simulink model "Complete_SAD_model"  (R2025b)
settings: Solver=ode4  StartTime=0.0  StopTime=10  FixedStep=0.01  RelTol=1e-3
values from neighbouring files (symbols this model uses):
  A = eye(3)    [Initial_condition.m]
  a_pink = exp(-2*pi*fc_pink*Ts_m*k_pink)    [Initial_condition.m]
  acc = deg2rad(0.5*randn)    [Initial_condition.m]
  Ap = eye(3)    [Initial_condition.m]
  D = 500*10^-12    (= 5e-10)    [Initial_condition.m]
  delay = 1    [Initial_condition.m]
  inv_Ir = inv(Ir)    [Initial_condition.m]
  Ir = diag([Irx,Iry,Irz])    [Initial_condition.m]
  J_B = diag([Ix,Iy,Iz])    [Initial_condition.m]
  m = [0.01; 0.01; 0.01]    [Initial_condition.m]
  m_max = [0.65; 0.65; 0.5]    [Initial_condition.m]
  Mr_max = [0.01; 0.01; 0.01]    [Initial_condition.m]
  mu_earth = 398600.433    [Initial_condition.m]
  mu_sun = 132712440017.987    (= 132712440018)    [Initial_condition.m]
  non_ort = deg2rad(-1+2*rand)    [Initial_condition.m]
  omega0 = [wx;wy;wz]    [Initial_condition.m]
  rES0_ECI = [0 AU 0]    [Initial_condition.m]
  seed = 0    [Initial_condition.m]
  sigma = (2*pi/60)/3    (= 0.0349065850399)    [Initial_condition.m]
  Ts_m = 1/f_m    (= 0.1)    [Initial_condition.m]
  Ts_ss = 1/f_ss    (= 0.1)    [Initial_condition.m]
  vES0_ECI = [(-sqrt(mu_sun/norm(rES0_ECI))) 0 0 ]    [Initial_condition.m]
  w_max = [250; 250; 250]    [Initial_condition.m]
undefined symbols (not defined in the file or in its folder): dspblkCoreblockFVToolHelper, gcbh, K, r0_ECI, v0_ECI
libraries: matrix_library x15, dspmathops x3, dspfdesign x3, vrlib x2
(part 1 of 3)
settings Model: Creator=Utente  LastModifiedBy=loren

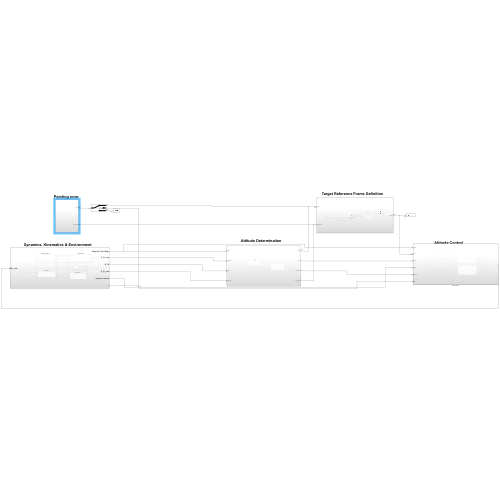
[thumbnail: Simulink's stored preview of the top-level diagram]
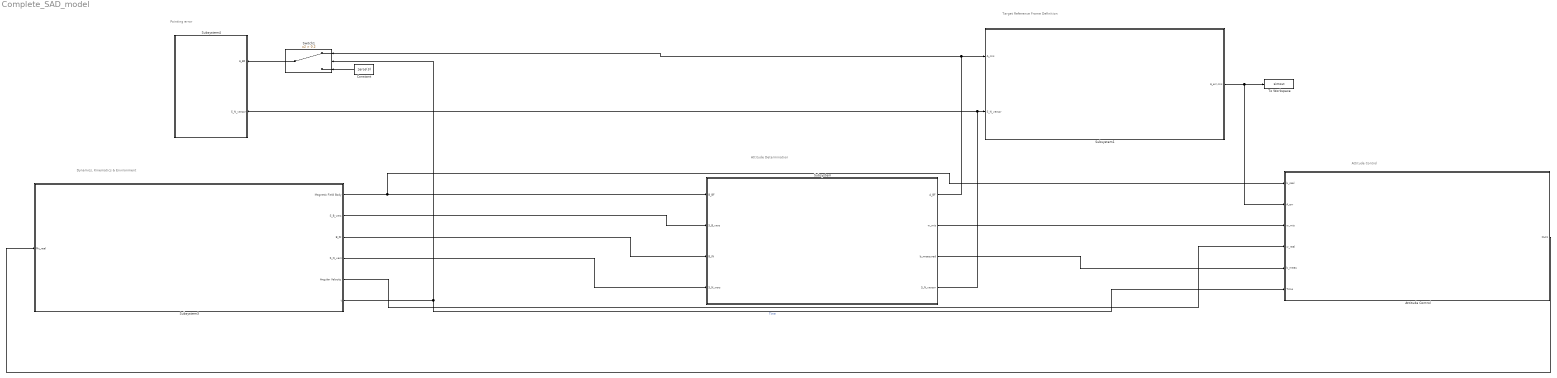
== system Complete_SAD_model ==
  note: Dynamics, Kinematics & Environment
  note: Attitude Determination
  note: Attitude Control
  note: Target Reference Frame Definition
  note: Pointing error
  Attitude Control : Subsystem
  Constant : Constant  Value=zeros(3)
  Subsystem : Subsystem
  Subsystem1 : Subsystem
  Subsystem3 : Subsystem
  Subsystem4 : Subsystem
  Switch1 : Switch  Criteria=u2 > Threshold  Threshold=0.2  SaturateOnIntegerOverflow=off  InputSameDT=off
  To Workspace : ToWorkspace  VariableName=simout  SaveFormat=Timeseries  SampleTime=-1
  wires:
  Subsystem3/1(Magnetic Field Body) -> Attitude Control/1(b_real), Subsystem/1(B_BF)
  Subsystem3/2(S_B_vers) -> Subsystem/2(S_B_vers)
  Subsystem3/3(B_IN) -> Subsystem/3(B_IN)
  Subsystem3/4(S_N_vers) -> Subsystem/4(S_N_vers)
  Subsystem/1(A_BF) -> Switch1/1, Subsystem1/1(A_mis)
  Subsystem/2(w_mis) -> Attitude Control/3(w_mis)
  Subsystem3/5(Angular Velocity) -> Attitude Control/4(w_real)
  Subsystem/3(b_measured) -> Attitude Control/5(b_meas)
  Subsystem3/6(t) -> Switch1/2, Attitude Control/6(Time)  "Time"
  Attitude Control/1(Out1) -> Subsystem3/1(Mc_real)
  Subsystem/4(S_N_versor) -> Subsystem4/2(S_N_versor), Subsystem1/2(S_N_versor)
  Subsystem1/1(A_err,mis) -> To Workspace/1, Attitude Control/2(A_err)
  Switch1/1 -> Subsystem4/1(A_BF)
  Constant/1 -> Switch1/3

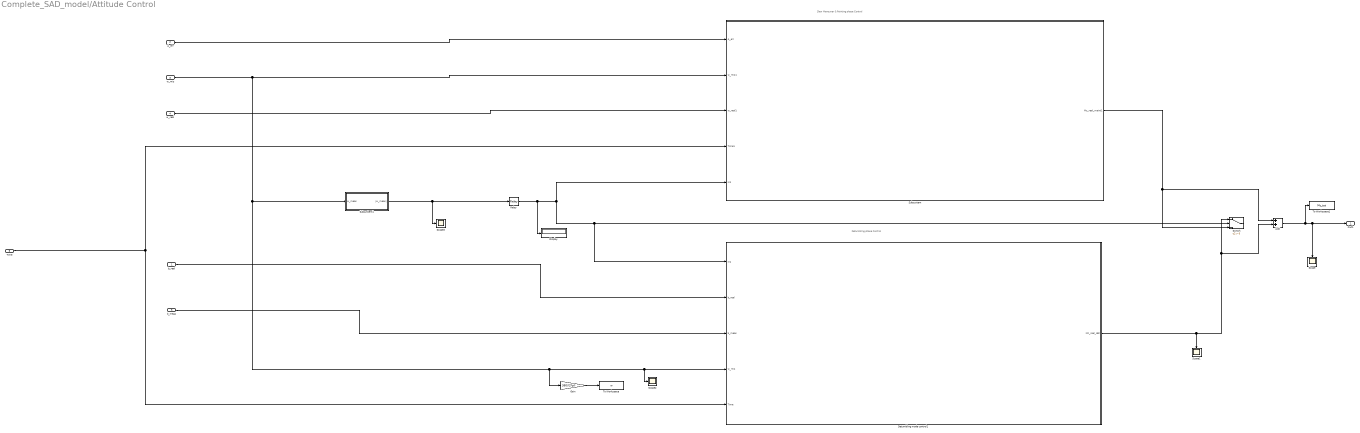
== system Complete_SAD_model/Attitude Control ==
  note: Detumbling phase Control
  note: Slew Manouver & Pointing phase Control
  b_real : Inport
  A_err : Inport  Port=2
  w_mis : Inport  Port=3
  w_real : Inport  Port=4
  b_meas : Inport  Port=5
  Time : Inport  Port=6
  Add : Sum
  Detumbling mode control1 : Subsystem
  Display : Display
  Gain : Gain  Gain=360/(2*pi)
  Relay : Relay  OnSwitchValue=0.15  OffSwitchValue=deg2rad(5)
  Scope{,1..3} (4 alike) : Scope
      Scope settings: ActiveDisplayYMinimum=-0.00066406553970955529  ActiveDisplayYMaximum=0.000676333066590346  DataLoggingVariableName=ScopeData20
      Scope1 settings: ActiveDisplayYMinimum=-0.000218043993955084  ActiveDisplayYMaximum=0.00024658945561407578  DataLoggingVariableName=ScopeData24
      Scope2 settings: ActiveDisplayYMinimum=-0.80919246331980188  ActiveDisplayYMaximum=0.81042984032750753  DataLoggingVariableName=ScopeData32
      Scope3 settings: ActiveDisplayYMinimum=0.021025794822100707  ActiveDisplayYMaximum=0.38469575455597654  DataLoggingVariableName=ScopeData37
  Subsystem : Subsystem
  Subsystem1 : Subsystem
  Switch : Switch  Criteria=u2 > Threshold  SaturateOnIntegerOverflow=off  InputSameDT=off
  To Workspace : ToWorkspace  VariableName=w  SaveFormat=Timeseries  SampleTime=-1
  To Workspace1 : ToWorkspace  VariableName=Mc_tot  SampleTime=-1
  Out1 : Outport
  wires:
  b_real/1 -> Detumbling mode control1/2(b_real)
  Detumbling mode control1/1(Mc_real_det) -> Scope1/1, Add/2, Switch/1
  Time/1 -> Subsystem/4(Time1), Detumbling mode control1/5(Time)
  b_meas/1 -> Detumbling mode control1/3(b_meas)
  w_mis/1 -> Subsystem1/1(w_meas), Gain/1, Scope2/1, Detumbling mode control1/4(w_mis), Subsystem/2(w_mis1)
  A_err/1 -> Subsystem/1(A_err)
  w_real/1 -> Subsystem/3(w_real1)
  Subsystem1/1(|w_meas|) -> Scope3/1, Relay/1
  Relay/1 -> Display/1, Subsystem/5(In1), Detumbling mode control1/1(In1), Switch/2
  Subsystem/1(Mc_real_maint1) -> Add/1, Switch/3
  Add/1 -> To Workspace1/1, Scope/1, Out1/1
  Gain/1 -> To Workspace/1

== system Complete_SAD_model/Subsystem ==
  note: Determination Algorithm
  note: Sensors
  B_BF : Inport
  S_B_vers : Inport  Port=2
  B_IN : Inport  Port=3
  S_N_vers : Inport  Port=4
  Determination Algorithm : Subsystem
  Scope : Scope
      settings: ActiveDisplayYMinimum=-1.125  ActiveDisplayYMaximum=0.12499999999999997  DataLoggingVariableName=ScopeData39
  Scope1 : Scope
      settings: ActiveDisplayYMinimum=-7.094188804581898E-5  ActiveDisplayYMaximum=5.8924288015728448E-5  DataLoggingVariableName=ScopeData40
  Subsystem2 : Subsystem
  A_BF : Outport
  w_mis : Outport  Port=2
  b_measured : Outport  Port=3
  S_N_versor : Outport  Port=4
  wires:
  S_B_vers/1 -> Subsystem2/2(S_B_vers)
  S_N_vers/1 -> Scope/1, S_N_versor/1, Determination Algorithm/4(S_N_vers)
  Subsystem2/1(b_measured) -> Determination Algorithm/2(b_measured), b_measured/1
  Determination Algorithm/1(A_BF) -> A_BF/1
  Subsystem2/2(S_B_measured) -> Determination Algorithm/1(S_B_measured)
  Determination Algorithm/2(w_mis) -> w_mis/1
  B_BF/1 -> Subsystem2/1(B_BF)
  B_IN/1 -> Scope1/1, Determination Algorithm/3(B_IN)

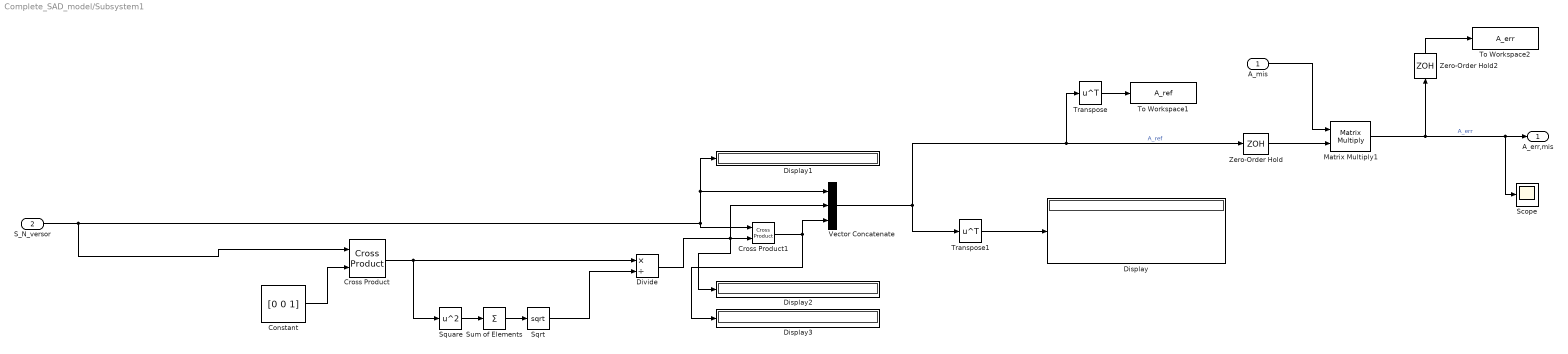
== system Complete_SAD_model/Subsystem1 ==
  A_mis : Inport
  S_N_versor : Inport  Port=2
  Constant : Constant  Value=[0 0 1]
  Cross Product : matrix_library/Cross Product
  Cross Product1 : matrix_library/Cross Product
  Display{,1..3} (4 alike) : Display
  Divide : Product  Inputs=*/
  Matrix Multiply1 : Product  Multiplication=Matrix(*)
  Scope : Scope
      settings: ActiveDisplayYMinimum=-1.0313451799509168  ActiveDisplayYMaximum=2.1593552960699949  DataLoggingVariableName=ScopeData36
  Sqrt : Sqrt
  Square : Math  Operator=square
  Sum of Elements : Sum  Inputs=+
  To Workspace1 : ToWorkspace  VariableName=A_ref  SampleTime=-1
  To Workspace2 : ToWorkspace  VariableName=A_err  SampleTime=-1
  Transpose : Math  Operator=transpose
  Transpose1 : Math  Operator=transpose
  Vector Concatenate : Concatenate  NumInputs=3  Mode=Multidimensional array  ConcatenateDimension=2
  Zero-Order Hold : ZeroOrderHold  SampleTime=0.1
  Zero-Order Hold2 : ZeroOrderHold  SampleTime=0.01
  A_err,mis : Outport
  wires:
  Square/1 -> Sum of Elements/1
  Zero-Order Hold/1 -> Matrix Multiply1/2
  Cross Product1/1 -> Vector Concatenate/3, Display3/1
  Sqrt/1 -> Divide/2
  Transpose/1 -> To Workspace1/1
  Matrix Multiply1/1 -> Zero-Order Hold2/1, Scope/1, A_err,mis/1  "A_err"
  Sum of Elements/1 -> Sqrt/1
  Vector Concatenate/1 -> Transpose1/1, Transpose/1, Zero-Order Hold/1  "A_ref"
  A_mis/1 -> Matrix Multiply1/1
  Zero-Order Hold2/1 -> To Workspace2/1
  Divide/1 -> Vector Concatenate/2, Display2/1, Cross Product1/2
  Cross Product/1 -> Divide/1, Square/1
  Constant/1 -> Cross Product/2
  S_N_versor/1 -> Cross Product/1, Vector Concatenate/1, Display1/1, Cross Product1/1
  Transpose1/1 -> Display/1

== system Complete_SAD_model/Subsystem3 ==
  note: Perturbations
  note: Dynamics
  note: Kinematics
  note: Orbit Propagation
  Mc_real : Inport
  " Attitude Dynamics" : Subsystem
  Attitude Kinematics  with orthonormalization : Subsystem
  Constant : Constant  Value=J_B
  Disturbance Torques : Subsystem
  Divide : Product  Inputs=*/
  MatrixMultiply : Product  Multiplication=Matrix(*)
  Orbita Propagation1 : Subsystem
  Scope : Scope
      settings: ActiveDisplayYMinimum=-0.0048523047678160009  ActiveDisplayYMaximum=0.00453129877837137  DataLoggingVariableName=ScopeData51
  Vector_Norm : Subsystem
  Magnetic Field Body : Outport
  S_B_vers : Outport  Port=2
  B_IN : Outport  Port=3
  S_N_vers : Outport  Port=4
  Angular Velocity : Outport  Port=5
  t : Outport  Port=6
  wires:
  Mc_real/1 -> " Attitude Dynamics"/3(Mc_real), Scope/1
  Disturbance Torques/4(t) -> t/1
  MatrixMultiply/1 -> S_B_vers/1
  Divide/1 -> MatrixMultiply/2, S_N_vers/1
  Vector_Norm/1(norm) -> Divide/2  "Position_Norm"
  Orbita Propagation1/4(r_SC/S) -> Vector_Norm/1(vector), Divide/1
  Disturbance Torques/3(B_IN) -> B_IN/1
  Disturbance Torques/2(Magnetic Field Body) -> Magnetic Field Body/1
  Attitude Kinematics  with orthonormalization/2(A_B | L) -> Disturbance Torques/5(A_B | L)
  Orbita Propagation1/2(h vector) -> Attitude Kinematics  with orthonormalization/3(h vector)
  Constant/1 -> Disturbance Torques/4("Matrix of Inertia "), " Attitude Dynamics"/1(Inertia Matrix)
  Orbita Propagation1/1("Norm of Position Spacecraft - Earth ") -> Disturbance Torques/1(Norm Position)
  Orbita Propagation1/3(Versore Posizione) -> Disturbance Torques/2(versore_Posizione), Attitude Kinematics  with orthonormalization/2(Versore Posizione)
  Disturbance Torques/1(Disturbance) -> " Attitude Dynamics"/2(Disturbo)
  " Attitude Dynamics"/1(Angular Velocity) -> Angular Velocity/1, Attitude Kinematics  with orthonormalization/1(Angular Velocity)
  Attitude Kinematics  with orthonormalization/1(Direction Cosine Matrix) -> MatrixMultiply/1, Disturbance Torques/3(DCM)

== system Complete_SAD_model/Subsystem4 ==
  A_BF : Inport
  S_N_versor : Inport  Port=2
  Acos : Trigonometry  Operator=acos
  Dot Product : DotProduct  OutDataTypeStr=Inherit: Inherit via internal rule
  Gain : Gain  Gain=360/(2*pi)
  Normalization : dspmathops/Normalization  NormType=2-norm  Bias=1e-10  NormOver=Each column  Dimension=1  roundingMode=Floor  overflowMode=off  accumDataTypeStr=Inherit: Same as product output  accumLastDataTypeStr=Inherit: Same as product output  outputDataTypeStr=Inherit: Same as product output  outputMin=[]  outputMax=[]  outputLastDataTypeStr=Inherit: Same as product output
  Normalization1 : dspmathops/Normalization  NormType=2-norm  Bias=1e-10  NormOver=Each column  Dimension=1  roundingMode=Floor  overflowMode=off  accumDataTypeStr=Inherit: Same as product output  accumLastDataTypeStr=Inherit: Same as product output  outputDataTypeStr=Inherit: Same as product output  outputMin=[]  outputMax=[]  outputLastDataTypeStr=Inherit: Same as product output
  Scope : Scope
      settings: ActiveDisplayYMinimum=-22.453635883732677  ActiveDisplayYMaximum=202.09419906568513  DataLoggingVariableName=ScopeData71
  Selector : Selector  NumberOfDimensions=2  InputPortWidth=3  IndexOptions=Index vector (dialog),Index vector (dialog)  Indices=1,1  OutputSizes=1,1
  Selector2 : Selector  NumberOfDimensions=2  InputPortWidth=3  IndexOptions=Index vector (dialog),Index vector (dialog)  Indices=1,2  OutputSizes=1,1
  Selector4 : Selector  NumberOfDimensions=2  InputPortWidth=3  IndexOptions=Index vector (dialog),Index vector (dialog)  Indices=1,3  OutputSizes=1,1
  To Workspace : ToWorkspace  VariableName=pointing_error  SampleTime=-1
  Vector Concatenate : Concatenate  NumInputs=3
  wires:
  Selector2/1 -> Vector Concatenate/2  "a12"
  Selector/1 -> Vector Concatenate/1  "a11"
  Selector4/1 -> Vector Concatenate/3  "a13"
  A_BF/1 -> Selector/1, Selector4/1, Selector2/1
  Vector Concatenate/1 -> Normalization1/1  "x_BF"
  S_N_versor/1 -> Normalization/1
  Normalization/1 -> Dot Product/1
  Normalization1/1 -> Dot Product/2
  Dot Product/1 -> Acos/1
  Acos/1 -> Gain/1
  Gain/1 -> Scope/1, To Workspace/1

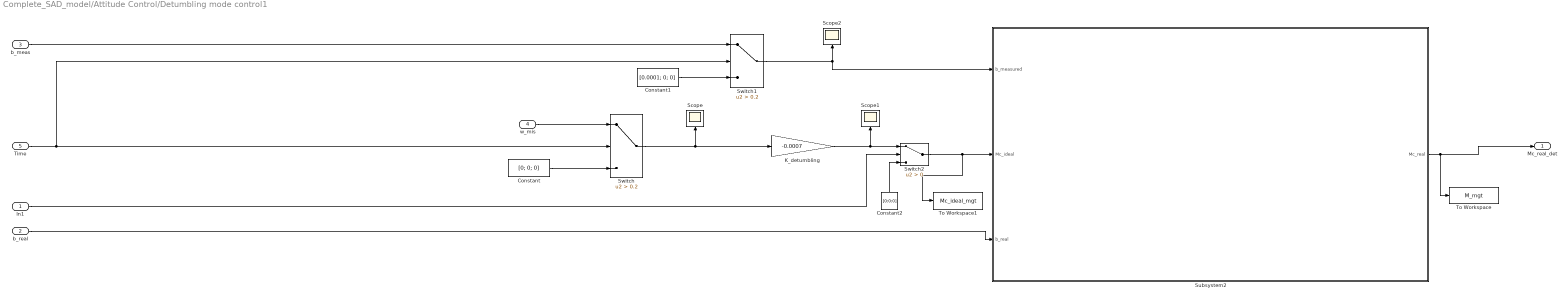
== system Complete_SAD_model/Attitude Control/Detumbling mode control1 ==
  In1 : Inport
  b_real : Inport  Port=2
  b_meas : Inport  Port=3
  w_mis : Inport  Port=4
  Time : Inport  Port=5
  Constant : Constant  Value=[0; 0; 0]
  Constant1 : Constant  Value=[0.0001; 0; 0]
  Constant2 : Constant  Value=[0;0;0]
  K_detumbling : Gain  Gain=-0.0007
  Scope : Scope
      settings: ActiveDisplayYMinimum=-0.83224888402197306  ActiveDisplayYMaximum=0.87185250448284746  DataLoggingVariableName=ScopeData3
  Scope1 : Scope
      settings: ActiveDisplayYMinimum=-0.001056362749452055  ActiveDisplayYMaximum=0.0010198107488302737  DataLoggingVariableName=ScopeData17
  Scope2 : Scope
      settings: ActiveDisplayYMinimum=-0.00021732143270324306  ActiveDisplayYMaximum=0.00011510450718215886  DataLoggingVariableName=ScopeData5
  Subsystem2 : Subsystem
  Switch : Switch  Criteria=u2 > Threshold  Threshold=0.2  SaturateOnIntegerOverflow=off  InputSameDT=off
  Switch1 : Switch  Criteria=u2 > Threshold  Threshold=0.2  SaturateOnIntegerOverflow=off  InputSameDT=off
  Switch2 : Switch  Criteria=u2 > Threshold  SaturateOnIntegerOverflow=off  InputSameDT=off
  To Workspace : ToWorkspace  VariableName=M_mgt  SampleTime=-1
  To Workspace1 : ToWorkspace  VariableName=Mc_ideal_mgt  SampleTime=-1
  Mc_real_det : Outport
  wires:
  b_meas/1 -> Switch1/1
  Constant/1 -> Switch/3
  Constant1/1 -> Switch1/3
  w_mis/1 -> Switch/1
  K_detumbling/1 -> Switch2/1, Scope1/1
  Switch1/1 -> Scope2/1, Subsystem2/1(b_measured)
  Switch/1 -> K_detumbling/1, Scope/1
  Time/1 -> Switch1/2, Switch/2
  b_real/1 -> Subsystem2/3(b_real)
  In1/1 -> Switch2/2
  Constant2/1 -> Switch2/3
  Switch2/1 -> To Workspace1/1, Subsystem2/2(Mc_ideal)
  Subsystem2/1(Mc_real) -> To Workspace/1, Mc_real_det/1

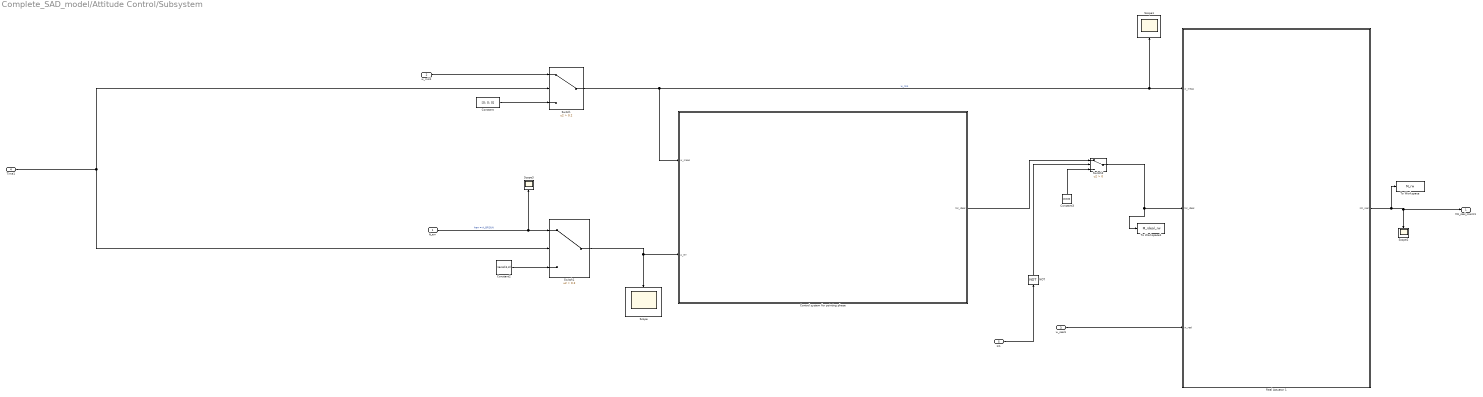
== system Complete_SAD_model/Attitude Control/Subsystem ==
  A_err : Inport
  w_mis1 : Inport  Port=2
  w_real1 : Inport  Port=3
  Time1 : Inport  Port=4
  In1 : Inport  Port=5
  Constant : Constant  Value=[0; 0; 0]
  Constant2 : Constant  Value=zeros(3,3)
  Constant3 : Constant  Value=[0;0;0]
  Control system for pointing phase : Subsystem
  NOT : Logic  Operator=NOT  IconShape=distinctive  AllPortsSameDT=off  OutDataTypeStr=boolean
  Real Actuator 1 : Subsystem
  Scope{,1..3} (4 alike) : Scope
      Scope settings: ActiveDisplayYMinimum=0.51490356419952588  ActiveDisplayYMaximum=1.1113602060789165  DataLoggingVariableName=ScopeData21
      Scope1 settings: ActiveDisplayYMinimum=-0.040624605457754565  ActiveDisplayYMaximum=0.040024288147769135  DataLoggingVariableName=ScopeData22
      Scope2 settings: ActiveDisplayYMinimum=-0.0019839698452016928  ActiveDisplayYMaximum=0.0020094703349881932  DataLoggingVariableName=ScopeData23
      Scope3 settings: DataLoggingVariableName=ScopeData28
  Switch : Switch  Criteria=u2 > Threshold  Threshold=0.2  SaturateOnIntegerOverflow=off  InputSameDT=off
  Switch1 : Switch  Criteria=u2 > Threshold  Threshold=0.2  SaturateOnIntegerOverflow=off  InputSameDT=off
  Switch2 : Switch  Criteria=u2 > Threshold  SaturateOnIntegerOverflow=off  InputSameDT=off
  To Workspace : ToWorkspace  VariableName=M_rw  SampleTime=-1
  To Workspace1 : ToWorkspace  VariableName=M_ideal_rw  SampleTime=-1
  Mc_real_maint1 : Outport
  wires:
  In1/1 -> NOT/1
  Time1/1 -> Switch1/2, Switch/2
  A_err/1 -> Switch1/1, Scope3/1  "Aerr = A_BF/SUN"
  Constant/1 -> Switch/3
  w_real1/1 -> Real Actuator 1/3(w_real)
  Switch1/1 -> Scope/1, Control system for pointing phase/2(A_err)
  w_mis1/1 -> Switch/1
  Switch/1 -> Real Actuator 1/1(w_meas), Scope1/1, Control system for pointing phase/1(w_meas)  "w_mis"
  Constant2/1 -> Switch1/3
  Control system for pointing phase/1(Mc_ideal) -> Switch2/1
  NOT/1 -> Switch2/2
  Constant3/1 -> Switch2/3
  Switch2/1 -> To Workspace1/1, Real Actuator 1/2(Mc_ideal)
  Real Actuator 1/1(Mc_real) -> To Workspace/1, Mc_real_maint1/1, Scope2/1

== system Complete_SAD_model/Attitude Control/Subsystem1 ==
  w_meas : Inport
  Sqrt : Sqrt
  Square : Math  Operator=square
  Sum of Elements : Sum  Inputs=+
  |w_meas| : Outport
  wires:
  w_meas/1 -> Square/1
  Sqrt/1 -> |w_meas|/1
  Square/1 -> Sum of Elements/1
  Sum of Elements/1 -> Sqrt/1

== system Complete_SAD_model/Subsystem/Determination Algorithm ==
  S_B_measured : Inport
  b_measured : Inport  Port=2
  B_IN : Inport  Port=3
  S_N_vers : Inport  Port=4
  ALGEBRAIC METHOD for ATTITUDE DETERMINATION 1 : Subsystem
  Angular velocity determination1 : Subsystem
  Scope{,1..5} (6 alike) : Scope
      Scope settings: ActiveDisplayYMinimum=-1  ActiveDisplayYMaximum=1  DataLoggingVariableName=ScopeData53
      Scope1 settings: ActiveDisplayYMinimum=-2.7577259976289361  ActiveDisplayYMaximum=2.8520572470875512  DataLoggingVariableName=ScopeData57
      Scope2 settings: DataLoggingVariableName=ScopeData58
      Scope3 settings: DataLoggingVariableName=ScopeData59
      Scope4 settings: DataLoggingVariableName=ScopeData60
      Scope5 settings: DataLoggingVariableName=ScopeData61
  A_BF : Outport
  w_mis : Outport  Port=2
  wires:
  ALGEBRAIC METHOD for ATTITUDE DETERMINATION 1/1(A_mis) -> A_BF/1, Scope/1, Angular velocity determination1/1(A_mis)  "A_BF"
  S_B_measured/1 -> Scope4/1, ALGEBRAIC METHOD for ATTITUDE DETERMINATION 1/2(S_B_measured)
  S_N_vers/1 -> Scope2/1, ALGEBRAIC METHOD for ATTITUDE DETERMINATION 1/4(S_N_vers)
  B_IN/1 -> Scope3/1, ALGEBRAIC METHOD for ATTITUDE DETERMINATION 1/3(B_IN)
  Angular velocity determination1/1(w_mis) -> Scope1/1, w_mis/1  "w_mis"
  b_measured/1 -> Scope5/1, ALGEBRAIC METHOD for ATTITUDE DETERMINATION 1/1(b_measured)

== system Complete_SAD_model/Subsystem/Subsystem2 ==
  note: Magnetometer
  note: Sun Sensor
  B_BF : Inport
  S_B_vers : Inport  Port=2
  MAGNETOMETER : Subsystem
  SUN SENSOR : Subsystem
      settings: PortSchema="{\"entries\":[{\"content\":{\"sides\":[{\"content\":{\"connectorIds\":[\"In1\"]},\"type\":\"ConnectorPlacement.EquallySpacedRectSide\",\"uuid\":\"3307fc53-f976-44c0-b732-30d51e7de2d2\"},{\"content\":{\"connectorIds\":[\"Out1\"],\"side\":\"RIGHT\"},\"type\":\"ConnectorPlacement.EquallySpacedRectSide\",\"uuid\":\"dd005eaf-9f48-4a06-9a65-62dab91bec2a\"},{\"content\":{\"side\":\"TOP\"},\"type\":\"ConnectorPlacement.EquallySpacedRectSide\",\"uuid\":\"b87f2816-b76f-4367-9475-2b3209047cf2\"},{\"content\":{\"connectorIds\":[\"Out2\"],\"side\":\"BOTTOM\"},\"type\":\"ConnectorPlacement.EquallySpacedRectSide\",\"uuid\":\"f1acf421-c567-4b56-8ca9-be9bc34615ea\"}]},\"type\":\"ConnectorPlacement.EquallySpacedConnector\",\"uuid\":\"0af9b085-f877-4503-8798-90c3da9edf65\"}],\"packageUris\":[\"http://schema.mathworks.com/mf0/Connector/R2020b\"],\"version\":\"1.0\"}"
  b_measured : Outport
  S_B_measured : Outport  Port=2
  wires:
  S_B_vers/1 -> SUN SENSOR/1(S_B_vers)
  B_BF/1 -> MAGNETOMETER/1(B_BF)
  SUN SENSOR/1(S_B_measured) -> S_B_measured/1
  MAGNETOMETER/1(b_measured) -> b_measured/1

== system Complete_SAD_model/Subsystem3/ Attitude Dynamics ==
  Inertia Matrix : Inport
  Disturbo : Inport  Port=2
  Mc_real : Inport  Port=3
  Add : Sum  Inputs=+++
  Cross Product : matrix_library/Cross Product
  Gain : Gain  Gain=inv(J_B)  Multiplication=Matrix(K*u)
  Integrator : Integrator  InitialCondition=omega0
  Product : Product  Multiplication=Matrix(*)
  Scope : Scope
      settings: ActiveDisplayYMinimum=-1  ActiveDisplayYMaximum=1  DataLoggingVariableName=ScopeData25
  Scope1 : Scope
      settings: ActiveDisplayYMinimum=-1  ActiveDisplayYMaximum=1  DataLoggingVariableName=ScopeData26
  Scope2 : Scope
      settings: ActiveDisplayYMinimum=-1  ActiveDisplayYMaximum=1  DataLoggingVariableName=ScopeData27
  To Workspace : ToWorkspace  VariableName=omega  SampleTime=-1
  Angular Velocity : Outport
  wires:
  Mc_real/1 -> Add/1
  Add/1 -> Gain/1
  Disturbo/1 -> Scope/1, Add/2
  Integrator/1 -> Scope2/1, Product/2, Cross Product/2, Angular Velocity/1, To Workspace/1  "Angular Velocity"
  Inertia Matrix/1 -> Product/1
  Gain/1 -> Integrator/1  "Angular Acceleration"
  Product/1 -> Cross Product/1  "I * w"
  Cross Product/1 -> Scope1/1, Add/3  "I * w x w"

== system Complete_SAD_model/Subsystem3/Attitude Kinematics  with orthonormalization ==
  Angular Velocity : Inport
  Versore Posizione : Inport  Port=2
  h vector : Inport  Port=3
  A_B|N : Subsystem
  A_L|N : Subsystem
  Product2 : Product  Multiplication=Matrix(*)
  Scope : Scope
      settings: ActiveDisplayYMinimum=-1.7642714488626539  ActiveDisplayYMaximum=1.9293671606099971  DataLoggingVariableName=ScopeData48
  Scope1 : Scope
      settings: ActiveDisplayYMinimum=-0.52373519233306431  ActiveDisplayYMaximum=0.98375738876943786  DataLoggingVariableName=ScopeData49
  Scope2 : Scope
      settings: DataLoggingVariableName=ScopeData50
  Transpose : Math  Operator=transpose
  Direction Cosine Matrix : Outport
  A_B | L : Outport  Port=2
  wires:
  Product2/1 -> Scope2/1, A_B | L/1  "A_B|L"
  h vector/1 -> A_L|N/2(h vector)
  Versore Posizione/1 -> A_L|N/1(Versore Posizione)
  Angular Velocity/1 -> A_B|N/1(Angular Velocity)
  Transpose/1 -> Scope/1, Product2/2  "A_L|N trasposta"
  A_B|N/1(Direction Cosine Matrix) -> Scope1/1, Product2/1, Direction Cosine Matrix/1  "A_B|N"
  A_L|N/1(A_L|N) -> Transpose/1  "A_L|N"

== system Complete_SAD_model/Subsystem3/Disturbance Torques ==
  note: Gravity Gradient
  note: Magnetic Field
  note: Drag
  Norm Position : Inport
  versore_Posizione : Inport  Port=2
  DCM : Inport  Port=3
  "Matrix of Inertia " : Inport  Port=4
  A_B | L : Inport  Port=5
  Add : Sum
  Gravity Gradient : Subsystem
  MAGNETIC FIELD PERTURBATION1 : Subsystem
  Scope : Scope
      settings: ActiveDisplayYMinimum=-2.9512104067111762E-7  ActiveDisplayYMaximum=3.7105496034992638E-7
  To Workspace : ToWorkspace  VariableName=Magnetic_Field_Body  SampleTime=-1
  To Workspace1 : ToWorkspace  VariableName=Magnetic_Torque  SampleTime=-1
  To Workspace2 : ToWorkspace  VariableName=gravity_torque  SampleTime=-1
  To Workspace3 : ToWorkspace  VariableName=Tot_disturbances  SampleTime=-1
  Disturbance : Outport
  Magnetic Field Body : Outport  Port=2
  B_IN : Outport  Port=3
  t : Outport  Port=4
  wires:
  Add/1 -> To Workspace3/1, Disturbance/1
  "Matrix of Inertia "/1 -> Gravity Gradient/1(Matrix of Inertia)
  A_B | L/1 -> Gravity Gradient/2(A_B | L)
  Gravity Gradient/1(Gravity Gradient Torque) -> Add/2, To Workspace2/1, Scope/1
  Norm Position/1 -> Gravity Gradient/3(Norm of Position), MAGNETIC FIELD PERTURBATION1/1(Norm_Position)
  versore_Posizione/1 -> MAGNETIC FIELD PERTURBATION1/2(versore_Posizione)
  DCM/1 -> MAGNETIC FIELD PERTURBATION1/3(DCM)
  MAGNETIC FIELD PERTURBATION1/1(Magnetique torque) -> Add/1, To Workspace1/1
  MAGNETIC FIELD PERTURBATION1/2(Magnetic Field Body) -> Magnetic Field Body/1, To Workspace/1
  MAGNETIC FIELD PERTURBATION1/3(B_IN) -> B_IN/1
  MAGNETIC FIELD PERTURBATION1/4(t) -> t/1

== system Complete_SAD_model/Subsystem3/Orbita Propagation1 ==
  " Earth - Sun Two - Body" : Subsystem
  Add : Sum
  Gain : Gain  Gain=-1
  Gain1 : Gain  Gain=-1
  Scope{1..6} (6 alike) : Scope
      Scope1 settings: ActiveDisplayYMinimum=-1.7011016377076345  ActiveDisplayYMaximum=1.6491374638547815  DataLoggingVariableName=ScopeData42
      Scope2 settings: ActiveDisplayYMinimum=-57600.130414773994  ActiveDisplayYMaximum=11329.241783614407  DataLoggingVariableName=ScopeData43
      Scope3 settings: ActiveDisplayYMinimum=6491.875025707579  ActiveDisplayYMaximum=6508.1247686317929  DataLoggingVariableName=ScopeData44
      Scope4 settings: ActiveDisplayYMinimum=-1.654875E+8  ActiveDisplayYMaximum=1.8387499999999996E+7  DataLoggingVariableName=ScopeData45
      Scope5 settings: ActiveDisplayYMinimum=-1.8037969949336094E+8  ActiveDisplayYMaximum=3.2487993679060951E+7  DataLoggingVariableName=ScopeData46
      Scope6 settings: ActiveDisplayYMinimum=-8118.4999742922937  ActiveDisplayYMaximum=8131.499768630646  DataLoggingVariableName=ScopeData47
  Spacecraft - Earth Two - Body : Subsystem
  To Workspace2 : ToWorkspace  VariableName=r_SATSUN_ECI  SampleTime=-1
  To Workspace3 : ToWorkspace  VariableName=r_SE_ECI  SampleTime=-1
  "Norm of Position Spacecraft - Earth " : Outport
  h vector : Outport  Port=2
  Versore Posizione : Outport  Port=3
  r_SC/S : Outport  Port=4
  wires:
  Spacecraft - Earth Two - Body/4(Versore Posizione) -> Scope1/1, Versore Posizione/1
  Gain1/1 -> Scope6/1, Add/1
  Gain/1 -> Scope4/1, To Workspace3/1, Add/2  "r_SE_ECI"
  Spacecraft - Earth Two - Body/1(Position Spacecraft .- Earth) -> Gain1/1  "r_ECI"
  Spacecraft - Earth Two - Body/3(h vector) -> Scope2/1, h vector/1
  Spacecraft - Earth Two - Body/2("Norm of Position Spacecraft - Earth ") -> Scope3/1, "Norm of Position Spacecraft - Earth "/1
  " Earth - Sun Two - Body"/1(Position Earth - Sun) -> Gain/1  "r_E/S"
  Add/1 -> To Workspace2/1, Scope5/1, r_SC/S/1  "r_SC/S"

== system Complete_SAD_model/Subsystem3/Vector_Norm ==
  vector : Inport
  Add : Sum  Inputs=+++
  Demux : Demux  Outputs=3
  Sqrt : Sqrt
  Square : Math  Operator=square
  Square1 : Math  Operator=square
  Square2 : Math  Operator=square
  norm : Outport
  wires:
  Sqrt/1 -> norm/1  "norm"
  Demux/2 -> Square1/1  "r_y"
  Add/1 -> Sqrt/1
  Square2/1 -> Add/3  "r_z^2"
  Demux/1 -> Square/1  "r_x"
  Demux/3 -> Square2/1  "r_z"
  Square1/1 -> Add/2  "r_y^2"
  Square/1 -> Add/1  "r_x^2"
  vector/1 -> Demux/1

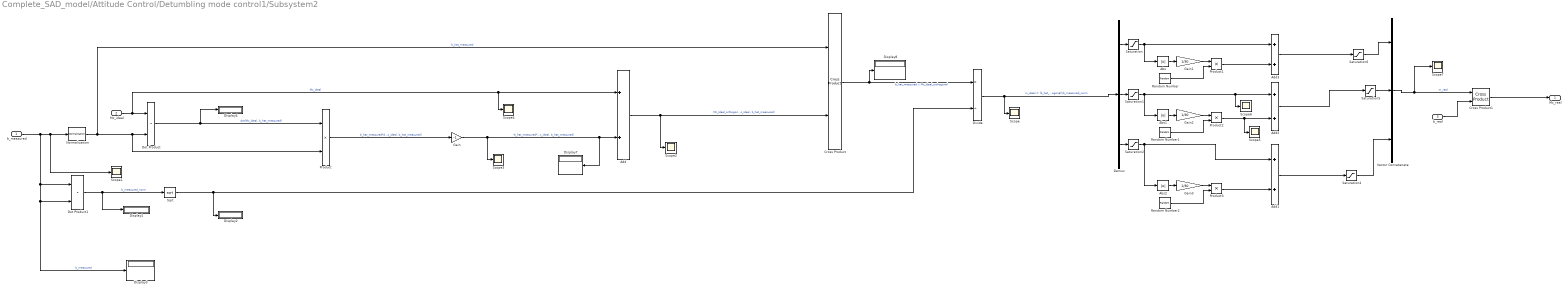
== system Complete_SAD_model/Attitude Control/Detumbling mode control1/Subsystem2 ==
  b_measured : Inport
  Mc_ideal : Inport  Port=2
  b_real : Inport  Port=3
  Abs : Abs  SaturateOnIntegerOverflow=off
  Abs1 : Abs  SaturateOnIntegerOverflow=off
  Abs2 : Abs  SaturateOnIntegerOverflow=off
  Add{,1..3} (4 alike) : Sum
  Cross Product : matrix_library/Cross Product
  Cross Product1 : matrix_library/Cross Product
  Demux : Demux  Outputs=3
  Display{1..4,7..8} (6 alike) : Display
  Divide : Product  Inputs=*/
  Dot Product : DotProduct  OutDataTypeStr=Inherit: Inherit via internal rule
  Dot Product1 : DotProduct  OutDataTypeStr=Inherit: Inherit via internal rule
  Gain : Gain  Gain=-1
  Gain1 : Gain  Gain=1/30
  Gain2 : Gain  Gain=1/30
  Gain3 : Gain  Gain=1/30
  Normalization : dspmathops/Normalization  NormType=2-norm  Bias=1e-10  NormOver=Each column  Dimension=1  roundingMode=Floor  overflowMode=off  accumDataTypeStr=Inherit: Same as product output  accumLastDataTypeStr=Inherit: Same as product output  outputDataTypeStr=Inherit: Same as product output  outputMin=[]  outputMax=[]  outputLastDataTypeStr=Inherit: Same as product output
  Product{,1..3} (4 alike) : Product
  Random Number : RandomNumber  SampleTime=0.01
  Random Number1 : RandomNumber  SampleTime=0.01
  Random Number2 : RandomNumber  SampleTime=0.01
  Saturation : Saturate  UpperLimit=m_max(1)  LowerLimit=-m_max(1)
  Saturation1 : Saturate  UpperLimit=m_max(2)  LowerLimit=-m_max(2)
  Saturation2 : Saturate  UpperLimit=m_max(3)  LowerLimit=-m_max(3)
  Saturation4 : Saturate  UpperLimit=m_max(3)  LowerLimit=-m_max(3)
  Saturation5 : Saturate  UpperLimit=m_max(2)  LowerLimit=-m_max(2)
  Saturation6 : Saturate  UpperLimit=m_max(1)  LowerLimit=-m_max(1)
  Scope{,1..7} (8 alike) : Scope
      Scope settings: ActiveDisplayYMinimum=-21.614327954012463  ActiveDisplayYMaximum=26.461567075211466  DataLoggingVariableName=ScopeData4
      Scope1 settings: ActiveDisplayYMinimum=-1  ActiveDisplayYMaximum=1  DataLoggingVariableName=ScopeData29
      Scope2 settings: ActiveDisplayYMinimum=-1  ActiveDisplayYMaximum=1  DataLoggingVariableName=ScopeData30
      Scope3 settings: ActiveDisplayYMinimum=-0.0092617354091048681  ActiveDisplayYMaximum=0.0064651724669457632  DataLoggingVariableName=ScopeData10
      Scope4 settings: ActiveDisplayYMinimum=-0.0037680920145246291  ActiveDisplayYMaximum=0.0021324597213686629  DataLoggingVariableName=ScopeData31
      Scope5 settings: ActiveDisplayYMinimum=-0.094525131302334545  ActiveDisplayYMaximum=0.093285625152668056  DataLoggingVariableName=ScopeData34
      Scope6 settings: ActiveDisplayYMinimum=-0.8125  ActiveDisplayYMaximum=0.8125  DataLoggingVariableName=ScopeData35
      Scope7 settings: ActiveDisplayYMinimum=-0.8125  ActiveDisplayYMaximum=0.8125  DataLoggingVariableName=ScopeData33
  Sqrt : Sqrt
  Vector Concatenate : Concatenate  NumInputs=3
  Mc_real : Outport
  wires:
  Cross Product1/1 -> Mc_real/1
  Vector Concatenate/1 -> Scope7/1, Cross Product1/1  "m_real"
  Dot Product1/1 -> Sqrt/1, Display1/1  "b_measured_norm"
  Divide/1 -> Demux/1, Scope/1  "m_ideal = (b_hat_measured x Mc_ideal_orthogonal)/b_measured_norm"
  Cross Product/1 -> Divide/1, Display8/1  "b_hat_measured x Mc_ideal_orthogonal"
  Add/1 -> Cross Product/2, Scope2/1  "Mc_ideal_orthogonal = Mc_ideal - b_hat_measured*dot(Mc_ideal, b_hat_measured)"
  Gain/1 -> Add/2, Display7/1, Scope3/1  "-b_hat_measured*dot(Mc_ideal, b_hat_measured)"
  Product/1 -> Gain/1  "b_hat_measured*dot(Mc_ideal, b_hat_measured)"
  Dot Product/1 -> Product/1, Display4/1  "dot(Mc_ideal, b_hat_measured)"
  Mc_ideal/1 -> Dot Product/1, Add/1, Scope4/1  "Mc_ideal"
  Normalization/1 -> Cross Product/1, Dot Product/2, Product/2  "b_hat_measured"
  b_measured/1 -> Dot Product1/1, Dot Product1/2, Display3/1, Normalization/1, Scope1/1  "b_measured"
  Sqrt/1 -> Divide/2, Display2/1
  b_real/1 -> Cross Product1/2
  Saturation1/1 -> Abs1/1, Scope6/1, Add2/1
  Demux/3 -> Saturation2/1
  Abs/1 -> Gain1/1
  Add3/1 -> Saturation6/1
  Random Number/1 -> Product1/2
  Random Number1/1 -> Product2/2
  Saturation2/1 -> Abs2/1, Add1/1
  Add2/1 -> Saturation5/1
  Demux/1 -> Saturation/1
  Demux/2 -> Saturation1/1
  Add1/1 -> Saturation4/1
  Gain3/1 -> Product3/1
  Gain1/1 -> Product1/1
  Saturation6/1 -> Vector Concatenate/1
  Gain2/1 -> Product2/1
  Product2/1 -> Scope5/1, Add2/2
  Random Number2/1 -> Product3/2
  Product3/1 -> Add1/2
  Saturation/1 -> Abs/1, Add3/1
  Saturation4/1 -> Vector Concatenate/3
  Abs2/1 -> Gain3/1
  Saturation5/1 -> Vector Concatenate/2
  Product1/1 -> Add3/2
  Abs1/1 -> Gain2/1

== system Complete_SAD_model/Attitude Control/Subsystem/Control system for pointing phase ==
  w_meas : Inport
  A_err : Inport  Port=2
  Constant : Constant  Value=-K
  MatrixMultiply : Product  Multiplication=Matrix(*)
  Selector : Selector  NumberOfDimensions=2  InputPortWidth=3  IndexOptions=Index vector (dialog),Index vector (dialog)  Indices=2,3  OutputSizes=1,1
  Selector2 : Selector  NumberOfDimensions=2  InputPortWidth=3  IndexOptions=Index vector (dialog),Index vector (dialog)  Indices=3,1  OutputSizes=1,1
  Selector4 : Selector  NumberOfDimensions=2  InputPortWidth=3  IndexOptions=Index vector (dialog),Index vector (dialog)  Indices=1,2  OutputSizes=1,1
  Vector Concatenate : Concatenate  NumInputs=4
  Mc_ideal : Outport
  wires:
  Vector Concatenate/1 -> MatrixMultiply/2
  A_err/1 -> Selector4/1, Selector2/1, Selector/1
  Selector2/1 -> Vector Concatenate/2  "a31"
  w_meas/1 -> Vector Concatenate/4
  Selector/1 -> Vector Concatenate/1  "a23"
  Selector4/1 -> Vector Concatenate/3  "a12"
  Constant/1 -> MatrixMultiply/1
  MatrixMultiply/1 -> Mc_ideal/1

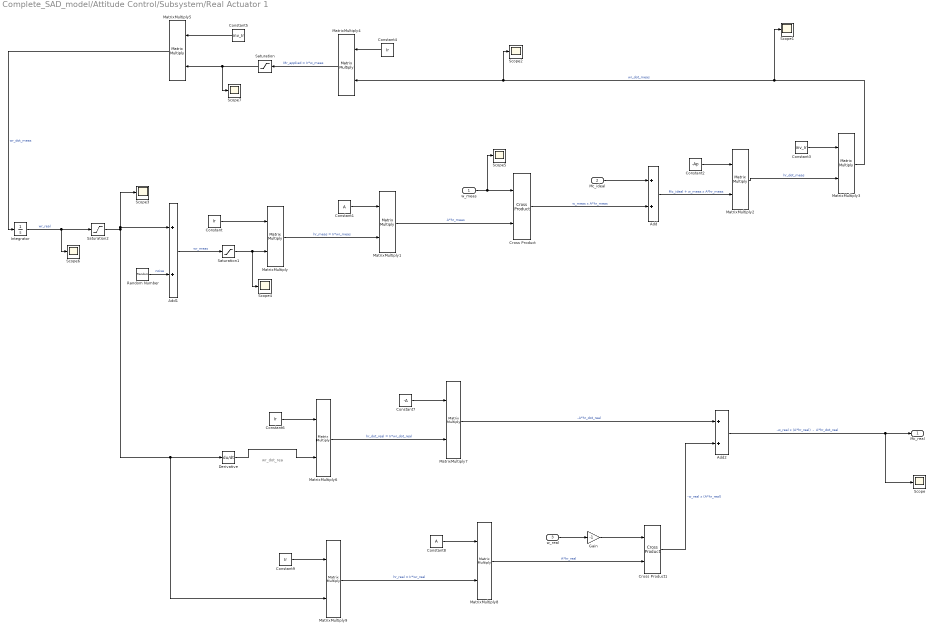
== system Complete_SAD_model/Attitude Control/Subsystem/Real Actuator 1 ==
  note: wr_dot_rea
  w_meas : Inport
  Mc_ideal : Inport  Port=2
  w_real : Inport  Port=3
  Add : Sum
  Add1 : Sum
  Add2 : Sum
  Constant{,4,6,9} (4 alike) : Constant  Value=Ir
  Constant1 : Constant  Value=A
  Constant2 : Constant  Value=-Ap
  Constant3 : Constant  Value=inv_Ir
  Constant5 : Constant  Value=inv_Ir
  Constant7 : Constant  Value=-A
  Constant8 : Constant  Value=A
  Cross Product : matrix_library/Cross Product
  Cross Product1 : matrix_library/Cross Product
  Derivative : Derivative
  Gain : Gain  Gain=-1
  Integrator : Integrator  InitialCondition=[0.02;0.02;0.02]
  MatrixMultiply{,1..9} (10 alike) : Product  Multiplication=Matrix(*)
  Random Number : RandomNumber  Variance=sigma^2  SampleTime=0.1
  Saturation : Saturate  UpperLimit=Mr_max  LowerLimit=-Mr_max
  Saturation1 : Saturate  UpperLimit=w_max  LowerLimit=-w_max
  Saturation2 : Saturate  UpperLimit=w_max  LowerLimit=-w_max
  Scope{,1..7} (8 alike) : Scope
      Scope settings: ActiveDisplayYMinimum=-0.0013388128325841997  ActiveDisplayYMaximum=0.0017880556064622005  DataLoggingVariableName=ScopeData4
      Scope1 settings: ActiveDisplayYMinimum=-26.40543979807255  ActiveDisplayYMaximum=275.8935317068225  DataLoggingVariableName=ScopeData5
      Scope2 settings: ActiveDisplayYMinimum=-273.56918829589108  ActiveDisplayYMaximum=342.86831435809211  DataLoggingVariableName=ScopeData6
      Scope3 settings: ActiveDisplayYMinimum=-59.282995533107886  ActiveDisplayYMaximum=58.310328732096352  DataLoggingVariableName=ScopeData7
      Scope4 settings: ActiveDisplayYMinimum=428.6194676671555  ActiveDisplayYMaximum=1088.2905548458557  DataLoggingVariableName=ScopeData10
      Scope5 settings: ActiveDisplayYMinimum=-0.13684680114496248  ActiveDisplayYMaximum=0.25965721191564439  DataLoggingVariableName=ScopeData15
      Scope6 settings: ActiveDisplayYMinimum=-50.174537610766144  ActiveDisplayYMaximum=32.89252642768961  DataLoggingVariableName=ScopeData19
      Scope7 settings: ActiveDisplayYMinimum=-0.014987318358616065  ActiveDisplayYMaximum=0.017939643357198422  DataLoggingVariableName=ScopeData38
  Mc_real : Outport
  wires:
  Saturation2/1 -> Add1/1, Scope3/1, Derivative/1, MatrixMultiply9/2
  Saturation1/1 -> MatrixMultiply/2, Scope4/1
  MatrixMultiply9/1 -> MatrixMultiply8/2  "hr_real = Ir*wr_real"
  Constant9/1 -> MatrixMultiply9/1
  Constant6/1 -> MatrixMultiply6/1
  w_real/1 -> Gain/1
  Add2/1 -> Scope/1, Mc_real/1  "-w_real x (A*hr_real)  -  A*hr_dot_real"
  MatrixMultiply8/1 -> Cross Product1/2  "A*hr_real"
  MatrixMultiply7/1 -> Add2/1  "-A*hr_dot_real"
  Constant8/1 -> MatrixMultiply8/1
  Constant7/1 -> MatrixMultiply7/1
  MatrixMultiply6/1 -> MatrixMultiply7/2  "hr_dot_real = Ir*wr_dot_real"
  Gain/1 -> Cross Product1/1
  Cross Product1/1 -> Add2/2  "-w_real x (A*hr_real)"
  Add1/1 -> Saturation1/1  "wr_meas"
  Random Number/1 -> Add1/2  "noise"
  MatrixMultiply5/1 -> Integrator/1  "wr_dot_meas"
  Constant5/1 -> MatrixMultiply5/1
  MatrixMultiply4/1 -> Saturation/1  "Mr_applied = Ir*w_meas"
  Constant4/1 -> MatrixMultiply4/1
  MatrixMultiply3/1 -> MatrixMultiply4/2, Scope2/1, Scope1/1  "wr_dot_meas"
  Constant3/1 -> MatrixMultiply3/1
  MatrixMultiply2/1 -> MatrixMultiply3/2  "hr_dot_meas"
  Constant2/1 -> MatrixMultiply2/1
  Add/1 -> MatrixMultiply2/2  "Mc_ideal + w_meas x A*hr_meas"
  Mc_ideal/1 -> Add/1
  Cross Product/1 -> Add/2  "w_meas x A*hr_meas"
  w_meas/1 -> Cross Product/1, Scope5/1
  MatrixMultiply1/1 -> Cross Product/2  "A*hr_meas"
  Constant1/1 -> MatrixMultiply1/1
  MatrixMultiply/1 -> MatrixMultiply1/2  "hr_meas = Ir*wr_meas"
  Constant/1 -> MatrixMultiply/1
  Integrator/1 -> Saturation2/1, Scope6/1  "wr_real"
  Derivative/1 -> MatrixMultiply6/2
  Saturation/1 -> Scope7/1, MatrixMultiply5/2

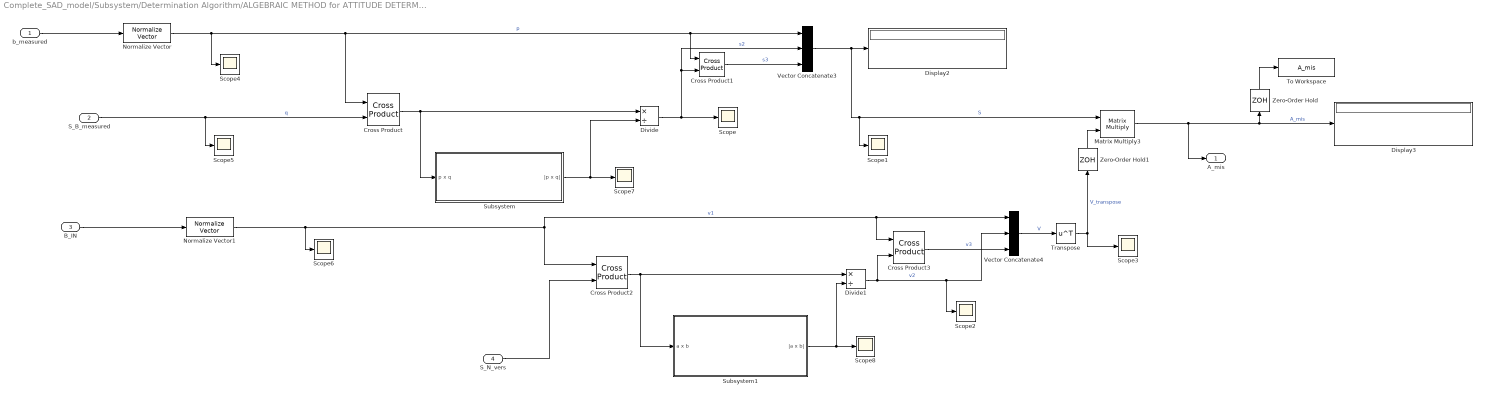
== system Complete_SAD_model/Subsystem/Determination Algorithm/ALGEBRAIC METHOD for ATTITUDE DETERMINATION 1 ==
  b_measured : Inport
  S_B_measured : Inport  Port=2
  B_IN : Inport  Port=3
  S_N_vers : Inport  Port=4
  Cross Product{,1..3} (4 alike) : matrix_library/Cross Product
  Display2 : Display
  Display3 : Display
  Divide : Product  Inputs=*/
  Divide1 : Product  Inputs=*/
  Matrix Multiply3 : Product  Multiplication=Matrix(*)
  Normalize Vector : vrlib/Utilities/Normalize Vector  maxzero=0
  Normalize Vector1 : vrlib/Utilities/Normalize Vector  maxzero=0
  Scope{,1..8} (9 alike) : Scope
      Scope settings: ActiveDisplayYMinimum=-1  ActiveDisplayYMaximum=1  DataLoggingVariableName=ScopeData62
      Scope1 settings: ActiveDisplayYMinimum=-1  ActiveDisplayYMaximum=1  DataLoggingVariableName=ScopeData63
      Scope2 settings: ActiveDisplayYMinimum=-1  ActiveDisplayYMaximum=1  DataLoggingVariableName=ScopeData64
      Scope3 settings: ActiveDisplayYMinimum=-0.85058331288263211  ActiveDisplayYMaximum=0.84151507814877036  DataLoggingVariableName=ScopeData65
      Scope4 settings: ActiveDisplayYMinimum=-1  ActiveDisplayYMaximum=1  DataLoggingVariableName=ScopeData66
      Scope5 settings: ActiveDisplayYMinimum=-1  ActiveDisplayYMaximum=1  DataLoggingVariableName=ScopeData67
      Scope6 settings: ActiveDisplayYMinimum=-1  ActiveDisplayYMaximum=1  DataLoggingVariableName=ScopeData68
      Scope7 settings: ActiveDisplayYMinimum=-1  ActiveDisplayYMaximum=1  DataLoggingVariableName=ScopeData69
      Scope8 settings: ActiveDisplayYMinimum=-0.45457430165202484  ActiveDisplayYMaximum=0.89352494006989025  DataLoggingVariableName=ScopeData70
  Subsystem : Subsystem
  Subsystem1 : Subsystem
  To Workspace : ToWorkspace  VariableName=A_mis  SampleTime=-1
  Transpose : Math  Operator=transpose
  Vector Concatenate3 : Concatenate  NumInputs=3  Mode=Multidimensional array  ConcatenateDimension=2
  Vector Concatenate4 : Concatenate  NumInputs=3  Mode=Multidimensional array  ConcatenateDimension=2
  Zero-Order Hold : ZeroOrderHold  SampleTime=0.01
  Zero-Order Hold1 : ZeroOrderHold  SampleTime=0.1
  A_mis : Outport
  wires:
  Zero-Order Hold1/1 -> Matrix Multiply3/2
  Subsystem1/1(|a x b|) -> Scope8/1, Divide1/2
  Subsystem/1(|p x q|) -> Scope7/1, Divide/2
  Zero-Order Hold/1 -> To Workspace/1
  Matrix Multiply3/1 -> Zero-Order Hold/1, Display3/1, A_mis/1  "A_mis"
  B_IN/1 -> Normalize Vector1/1
  Cross Product3/1 -> Vector Concatenate4/3  "v3"
  S_N_vers/1 -> Cross Product2/2
  Transpose/1 -> Scope3/1, Zero-Order Hold1/1  "V_transpose"
  Normalize Vector1/1 -> Scope6/1, Cross Product3/1, Vector Concatenate4/1, Cross Product2/1  "v1"
  Vector Concatenate4/1 -> Transpose/1  "V"
  b_measured/1 -> Normalize Vector/1
  Normalize Vector/1 -> Scope4/1, Vector Concatenate3/1, Cross Product1/1, Cross Product/1  "p"
  S_B_measured/1 -> Scope5/1, Cross Product/2  "q"
  Cross Product1/1 -> Vector Concatenate3/3  "s3"
  Divide1/1 -> Cross Product3/2, Scope2/1, Vector Concatenate4/2  "v2"
  Vector Concatenate3/1 -> Display2/1, Scope1/1, Matrix Multiply3/1  "S"
  Cross Product2/1 -> Divide1/1, Subsystem1/1(a x b)
  Cross Product/1 -> Divide/1, Subsystem/1(p x q)
  Divide/1 -> Scope/1, Vector Concatenate3/2, Cross Product1/2  "s2"

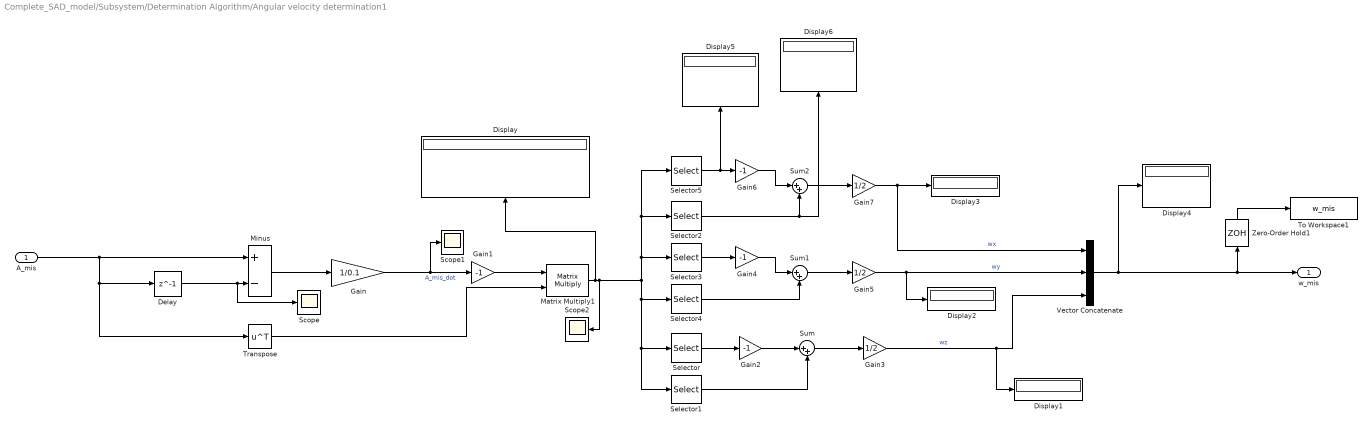
== system Complete_SAD_model/Subsystem/Determination Algorithm/Angular velocity determination1 ==
  A_mis : Inport
  Delay : Delay  DelayLength=1  SampleTime=0.1
  Display{,1..6} (7 alike) : Display
  Gain : Gain  Gain=1/0.1
  Gain{1..2,4,6} (4 alike) : Gain  Gain=-1
  Gain3 : Gain  Gain=1/2
  Gain5 : Gain  Gain=1/2
  Gain7 : Gain  Gain=1/2
  Matrix Multiply1 : Product  Multiplication=Matrix(*)
  Minus : Sum  Inputs=+-
  Scope : Scope
      settings: DataLoggingVariableName=ScopeData54
  Scope1 : Scope
      settings: DataLoggingVariableName=ScopeData55
  Scope2 : Scope
      settings: DataLoggingVariableName=ScopeData56
  Selector : Selector  NumberOfDimensions=2  InputPortWidth=3  IndexOptions=Index vector (dialog),Index vector (dialog)  Indices=1,2  OutputSizes=1,1
  Selector1 : Selector  NumberOfDimensions=2  InputPortWidth=3  IndexOptions=Index vector (dialog),Index vector (dialog)  Indices=2,1  OutputSizes=1,1
  Selector2 : Selector  NumberOfDimensions=2  InputPortWidth=3  IndexOptions=Index vector (dialog),Index vector (dialog)  Indices=3,2  OutputSizes=1,1
  Selector3 : Selector  NumberOfDimensions=2  InputPortWidth=3  IndexOptions=Index vector (dialog),Index vector (dialog)  Indices=3,1  OutputSizes=1,1
  Selector4 : Selector  NumberOfDimensions=2  InputPortWidth=3  IndexOptions=Index vector (dialog),Index vector (dialog)  Indices=1,3  OutputSizes=1,1
  Selector5 : Selector  NumberOfDimensions=2  InputPortWidth=3  IndexOptions=Index vector (dialog),Index vector (dialog)  Indices=2,3  OutputSizes=1,1
  Sum : Sum  Inputs=|++
  Sum1 : Sum  Inputs=|++
  Sum2 : Sum  Inputs=|++
  To Workspace1 : ToWorkspace  VariableName=w_mis  SampleTime=-1
  Transpose : Math  Operator=transpose
  Vector Concatenate : Concatenate  NumInputs=3
  Zero-Order Hold1 : ZeroOrderHold  SampleTime=0.01
  w_mis : Outport
  wires:
  Gain2/1 -> Sum/1
  Vector Concatenate/1 -> Display4/1, w_mis/1, Zero-Order Hold1/1
  Minus/1 -> Gain/1
  Zero-Order Hold1/1 -> To Workspace1/1
  Gain4/1 -> Sum1/1
  Selector/1 -> Gain2/1
  Sum2/1 -> Gain7/1
  Gain1/1 -> Matrix Multiply1/1
  Selector1/1 -> Sum/2
  Selector2/1 -> Sum2/2, Display6/1
  Gain5/1 -> Vector Concatenate/2, Display2/1  "wy"
  Sum1/1 -> Gain5/1
  Gain3/1 -> Display1/1, Vector Concatenate/3  "wz"
  Gain7/1 -> Vector Concatenate/1, Display3/1  "wx"
  Transpose/1 -> Matrix Multiply1/2
  Gain/1 -> Scope1/1, Gain1/1  "A_mis_dot"
  A_mis/1 -> Minus/1, Delay/1, Transpose/1
  Matrix Multiply1/1 -> Display/1, Scope2/1, Selector4/1, Selector/1, Selector1/1, Selector5/1, Selector2/1, Selector3/1
  Delay/1 -> Scope/1, Minus/2
  Selector5/1 -> Display5/1, Gain6/1
  Selector4/1 -> Sum1/2
  Selector3/1 -> Gain4/1
  Sum/1 -> Gain3/1
  Gain6/1 -> Sum2/1

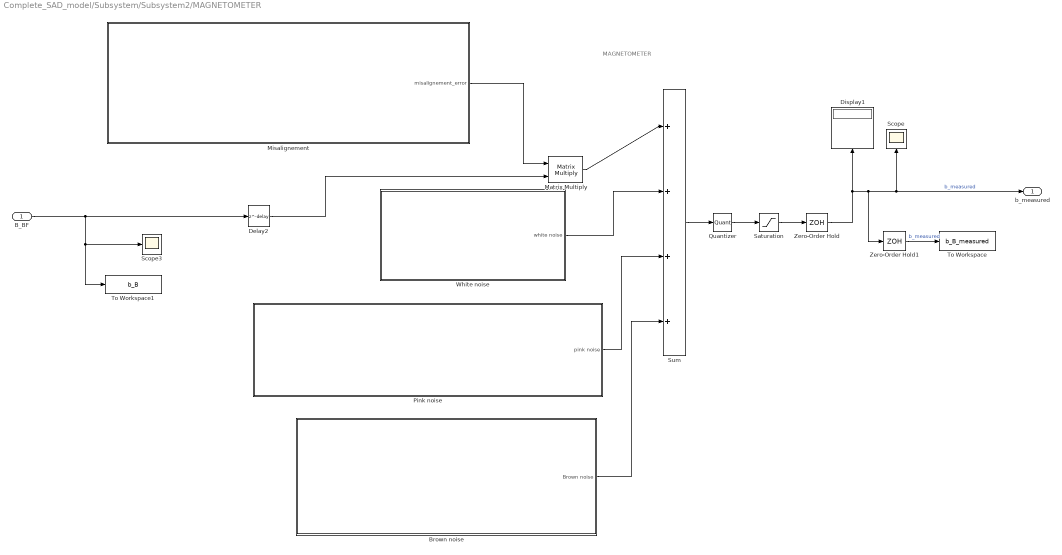
== system Complete_SAD_model/Subsystem/Subsystem2/MAGNETOMETER ==
  note: MAGNETOMETER
  B_BF : Inport
  Brown noise : Subsystem
  Delay2 : Delay  DelayLength=delay  InitialCondition=NaN  SampleTime=Ts_m
  Display1 : Display
  Matrix Multiply : Product  Multiplication=Matrix(*)
  Misalignement : Subsystem
  Pink noise : Subsystem
  Quantizer : Quantizer  QuantizationInterval=Res
  Saturation : Saturate  UpperLimit=50000  LowerLimit=-50000
  Scope : Scope
      settings: ActiveDisplayYMinimum=-0.0013517114012952852  ActiveDisplayYMaximum=0.0010059470701214873  DataLoggingVariableName=ScopeData8
  Scope3 : Scope
      settings: ActiveDisplayYMinimum=-52435.422682547833  ActiveDisplayYMaximum=70878.399240296567  DataLoggingVariableName=ScopeData12
  Sum : Sum  Inputs=|++++
  To Workspace : ToWorkspace  VariableName=b_B_measured  SampleTime=-1
  To Workspace1 : ToWorkspace  VariableName=b_B  SampleTime=-1
  White noise : Subsystem
  Zero-Order Hold : ZeroOrderHold  SampleTime=Ts_m
  Zero-Order Hold1 : ZeroOrderHold  SampleTime=0.01
  b_measured : Outport
  wires:
  Zero-Order Hold1/1 -> To Workspace/1  "b_measured"
  Delay2/1 -> Matrix Multiply/2
  B_BF/1 -> Scope3/1, To Workspace1/1, Delay2/1
  Brown noise/1(Brown noise) -> Sum/4
  Pink noise/1(pink noise) -> Sum/3
  White noise/1(white noise) -> Sum/2
  Misalignement/1(misalignement_error) -> Matrix Multiply/1
  Saturation/1 -> Zero-Order Hold/1
  Sum/1 -> Quantizer/1
  Matrix Multiply/1 -> Sum/1
  Quantizer/1 -> Saturation/1
  Zero-Order Hold/1 -> Display1/1, Zero-Order Hold1/1, Scope/1, b_measured/1  "b_measured"

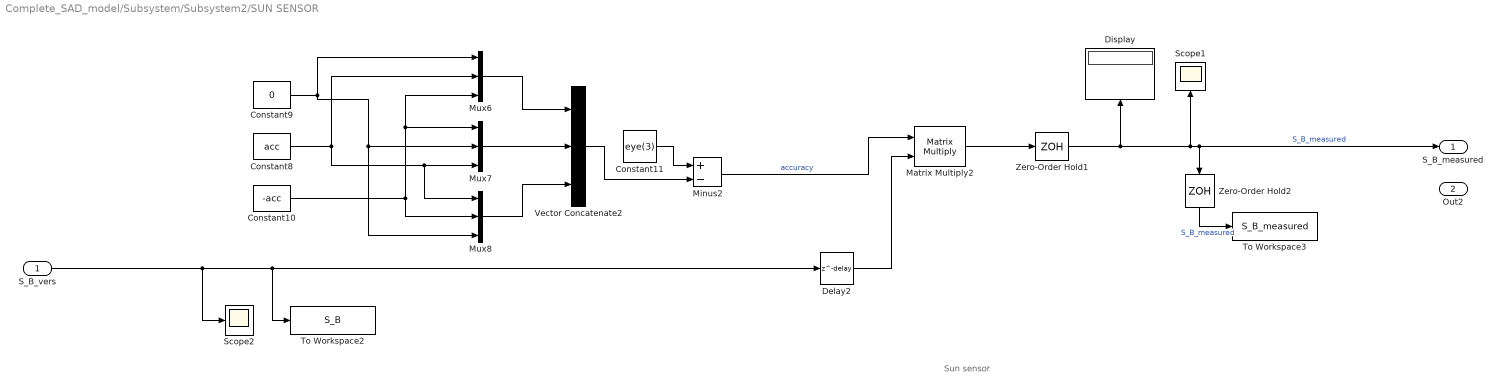
== system Complete_SAD_model/Subsystem/Subsystem2/SUN SENSOR ==
  note: Sun sensor
  S_B_vers : Inport
  Constant10 : Constant  Value=-acc
  Constant11 : Constant  Value=eye(3)
  Constant8 : Constant  Value=acc
  Constant9 : Constant  Value=0
  Delay2 : Delay  DelayLength=delay  InitialCondition=NaN  SampleTime=Ts_ss
  Display : Display
  Matrix Multiply2 : Product  Multiplication=Matrix(*)
  Minus2 : Sum  Inputs=+-
  Mux6 : Mux  Inputs=3
  Mux7 : Mux  Inputs=3
  Mux8 : Mux  Inputs=3
  Scope1 : Scope
      settings: ActiveDisplayYMinimum=-1.4960334523715215  ActiveDisplayYMaximum=1.5628617797695241  DataLoggingVariableName=ScopeData9
  Scope2 : Scope
      settings: ActiveDisplayYMinimum=-1  ActiveDisplayYMaximum=1  DataLoggingVariableName=ScopeData11
  To Workspace2 : ToWorkspace  VariableName=S_B  SampleTime=-1
  To Workspace3 : ToWorkspace  VariableName=S_B_measured  SampleTime=-1
  Vector Concatenate2 : Concatenate  NumInputs=3  Mode=Multidimensional array  ConcatenateDimension=2
  Zero-Order Hold1 : ZeroOrderHold  SampleTime=Ts_ss
  Zero-Order Hold2 : ZeroOrderHold  SampleTime=0.01
  S_B_measured : Outport
  Out2 : Outport  Port=2
  wires:
  Zero-Order Hold2/1 -> To Workspace3/1  "S_B_measured"
  Delay2/1 -> Matrix Multiply2/2
  S_B_vers/1 -> Scope2/1, Delay2/1, To Workspace2/1
  Mux7/1 -> Vector Concatenate2/2
  Constant8/1 -> Mux6/2, Mux7/3, Mux8/1
  Minus2/1 -> Matrix Multiply2/1  "accuracy"
  Constant10/1 -> Mux7/1, Mux6/3, Mux8/2
  Mux6/1 -> Vector Concatenate2/1
  Vector Concatenate2/1 -> Minus2/2
  Zero-Order Hold1/1 -> Display/1, Scope1/1, S_B_measured/1, Zero-Order Hold2/1  "S_B_measured"
  Constant9/1 -> Mux6/1, Mux7/2, Mux8/3
  Mux8/1 -> Vector Concatenate2/3
  Matrix Multiply2/1 -> Zero-Order Hold1/1
  Constant11/1 -> Minus2/1

== system Complete_SAD_model/Subsystem3/Attitude Kinematics  with orthonormalization/A_B|N ==
  Angular Velocity : Inport
  Add : Sum  Inputs=-+
  Constant1 : Constant  Value=0
  Demux : Demux  Outputs=3
  Gain{,1..3} (4 alike) : Gain  Gain=-1
  Gain4 : Gain  Gain=3/2
  Gain5 : Gain  Gain=1/2
  Integrator : Integrator  InitialCondition=eye(3)
  Math Function : Math  Operator=transpose
  Mux : Mux  Inputs=9
  Product : Product  Multiplication=Matrix(*)
  Product1 : Product  Inputs=3  Multiplication=Matrix(*)
  Reshape : Reshape  OutputDimensionality=Customize  OutputDimensions=[3,3]
  To Workspace : ToWorkspace  VariableName=DCM  SampleTime=-1
  Direction Cosine Matrix : Outport
  wires:
  Mux/1 -> Reshape/1
  Gain/1 -> Mux/8
  Demux/1 -> Mux/6, Gain/1  "wx"
  Product1/1 -> Add/1
  Gain1/1 -> Mux/3
  Constant1/1 -> Mux/5, Mux/9, Mux/1
  Demux/3 -> Mux/2, Gain2/1  "wz"
  Reshape/1 -> Gain3/1
  Math Function/1 -> Product1/2
  Demux/2 -> Mux/7, Gain1/1  "wy"
  Gain3/1 -> Product/1
  Gain5/1 -> Product1/1
  Angular Velocity/1 -> Demux/1
  Gain4/1 -> Add/2
  Product/1 -> Integrator/1  "dA"
  Integrator/1 -> Gain5/1, Math Function/1, Product1/3, Gain4/1, Direction Cosine Matrix/1, To Workspace/1  "DCM"
  Gain2/1 -> Mux/4
  Add/1 -> Product/2

== system Complete_SAD_model/Subsystem3/Attitude Kinematics  with orthonormalization/A_L|N ==
  Versore Posizione : Inport
  h vector : Inport  Port=2
  Cross Product : matrix_library/Cross Product
  Matrix Concatenate : Concatenate  NumInputs=3  Mode=Multidimensional array
  Product : Product  Inputs=*/
  Transpose : Math  Operator=transpose
  Transpose1 : Math  Operator=transpose
  Transpose2 : Math  Operator=transpose
  Vector_Norm : Subsystem
  A_L|N : Outport
  wires:
  Product/1 -> Transpose2/1, Cross Product/1  "h hat"
  Vector_Norm/1(norm) -> Product/2  "Norm"
  Matrix Concatenate/1 -> A_L|N/1
  Transpose1/1 -> Matrix Concatenate/2  "theta hat trasposto"
  Transpose2/1 -> Matrix Concatenate/3  "h hat trasposto"
  Transpose/1 -> Matrix Concatenate/1  "versore posizione trasposto"
  Cross Product/1 -> Transpose1/1  "theta hat"
  Versore Posizione/1 -> Cross Product/2, Transpose/1
  h vector/1 -> Vector_Norm/1(vector), Product/1

== system Complete_SAD_model/Subsystem3/Disturbance Torques/Gravity Gradient ==
  Matrix of Inertia : Inport
  A_B | L : Inport  Port=2
  Norm of Position : Inport  Port=3
  Constant : Constant  Value=3
  Constant1 : Constant  Value=[1;0;0]
  Cross Product : matrix_library/Cross Product
  Power : Math  Operator=pow
  Product : Product  Inputs=**/
  Product1 : Product  Multiplication=Matrix(*)
  Product2 : Product  Multiplication=Matrix(*)
  Product3 : Product
  Scope : Scope
      settings: ActiveDisplayYMinimum=-1  ActiveDisplayYMaximum=1  DataLoggingVariableName=ScopeData2
  mu_Earth : Constant  Value=mu_earth
  Gravity Gradient Torque : Outport
  wires:
  Power/1 -> Product/3
  Product1/1 -> Product2/2, Cross Product/1  "r_B"
  Constant1/1 -> Product1/2  "r_L"
  Product/1 -> Product3/1
  Constant/1 -> Power/2, Product/2
  A_B | L/1 -> Product1/1
  Product2/1 -> Cross Product/2
  mu_Earth/1 -> Product/1
  Product3/1 -> Gravity Gradient Torque/1
  Norm of Position/1 -> Power/1, Scope/1
  Cross Product/1 -> Product3/2
  Matrix of Inertia/1 -> Product2/1
